simulink model "FM"  (R2023b)
settings: Solver=VariableStepAuto  StartTime=0.0  StopTime=10  RelTol=1e-3
libraries: commanapbnd3 x1
settings Model: Creator=lxl  LastModifiedBy=lxl

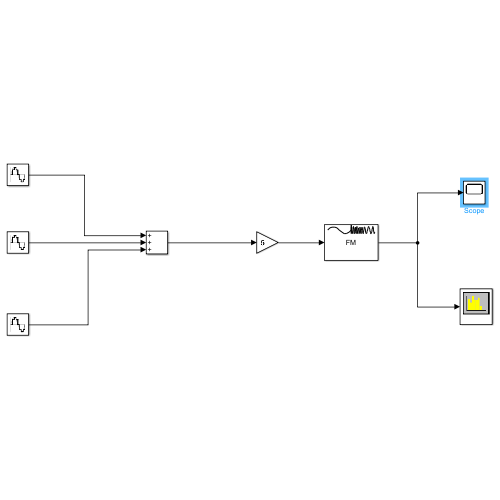
[thumbnail: Simulink's stored preview of the top-level diagram]
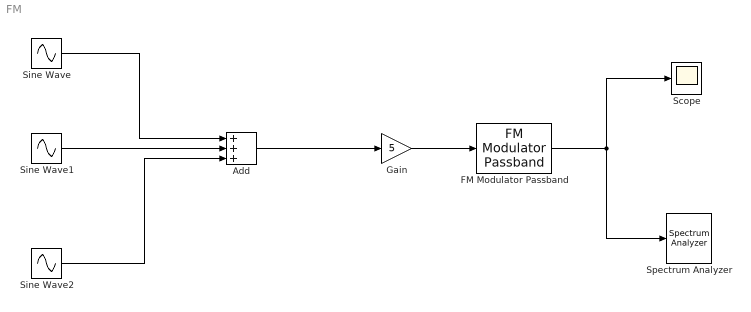
== system FM ==
  Add : Sum  Inputs=+++
  FM Modulator Passband : commanapbnd3/FM Modulator Passband  Fc=1000  Ph=0  Kc=50
  Gain : Gain  Gain=5
  Scope : Scope
  Sine Wave : Sin  Amplitude=0.3  Frequency=2*pi*10  SampleTime=1/3000
  Sine Wave1 : Sin  Amplitude=0.2  Frequency=2*pi*20  Phase=pi/6  SampleTime=1/3000
  Sine Wave2 : Sin  Amplitude=0.5  Frequency=2*pi*30  Phase=pi/3  SampleTime=1/3000
  Spectrum Analyzer : SpectrumAnalyzer  WindowPosition=[368.000000,182.000000,800.000000,500.000000,]  ScopeFrameLocation=window  YLimits=[-66.74572258,21.31012559]
  wires:
  Sine Wave/1 -> Add/1
  Sine Wave1/1 -> Add/2
  Sine Wave2/1 -> Add/3
  Add/1 -> Gain/1
  Gain/1 -> FM Modulator Passband/1
  FM Modulator Passband/1 -> Scope/1, Spectrum Analyzer/1
